simulink model "KUKA_coupled"  (R2021b)
settings: Solver=ode4  StartTime=0.0  StopTime=0.01  FixedStep=0.01  RelTol=1e-3  EnableMultiTasking=on
InitFcn:
  | % ************** Initiate forces
  | % f0=[0;0;0;0;0;0];
  | % f0=[0;0;0;0;0;0;0];
  | %f_0=[0;0;0];
  | %f_m=[0;0];
  | %f_e=[0;0;0;0;0;0];
  | %iota0=eye(6);
  | % ************** Initiate states
  | %q_m=[2;1];
  | %q_dot_m=[0;1];
  | %P=[0;0;0];
  | %V_I0=[0;0;0];
  | % ************** Load main
  | %run(Main.m)
StopFcn:
  | %format long
  | %table(out.qddot.data(:,1)',out.qddot_ref.data(1,:))
values from neighbouring files (symbols this model uses):
  diag_M = diagonalize(M_frak0, M_frak)    [Create_Robot.m]    (also in Main.m; Main__iiwa7.m; diagonalize.m = zeros(6*(n+1),6*(n+1)); test_C_Main.m)
  f_0 = [0;0;0]    [Create_Robot.m]    (also in Main.m; Main__iiwa7.m = [0;0;0;0;0;0]; test_C_Main.m)
  f_e = [0;0;0;0;0;0]    [Create_Robot.m]    (also in Main.m = [0;0;0]; Main__iiwa7.m; test_C_Main.m)
  f_m = [0;0]    [Create_Robot.m]    (also in Main.m; Main__iiwa7.m; test_C_Main.m)
  I0 = eye(3)*416.667    [Create_Robot.m]    (also in Main.m; Main__iiwa7.m = eye(3)*1.66667; test_C_Main.m)
  iota0 = [1 0 0; 0 1 0;zeros(3,3);0 0 1]    [Create_Robot.m]    (also in Main.m = [1 0 0 0 0 0; 0 1 0 0 0 0; 0 0 0 0 0 1]'; Main__iiwa7.m = eye(6,6); test_C_Main.m)
  m0 = 100    [Create_Robot.m]    (also in Main.m; Main__iiwa7.m = 10; test_C_Main.m)
  P = [0;0;0]    [Create_Robot.m]    (also in Main.m = M0*V_I0+M0m*q_dot_m; Main__iiwa7.m = M0*V_I0+M0m*q_dot_m; test_C_Main.m)
  q_dot_m = [0;0]    [Create_Robot.m]    (also in Main.m; Main__iiwa7.m; test_C_Main.m)
  q_m = [0;0]    [Create_Robot.m]    (also in Main.m = [0.2;0.4]; Main__iiwa7.m = [0.2;0.4]; test_C_Main.m = [1;0])
  sc_size = 5    [Main.m]    (also in Main__iiwa7.m = 1)
  X = [0 -x(3) x(2) ; x(3) 0 -x(1) ; -x(2) x(1) 0 ]    [skewsym.m]
  Xi_m_matrix = zeros(6*n,n)    [Create_Robot.m]    (also in Main.m; Main__iiwa7.m; test_C_Main.m)
undefined symbols (not defined in the file or in its folder): rho_0t, V_0t, Xi_m, Y, Z
libraries: sm_lib x87, nesl_utility x51, robotcorelib x2
(part 2 of 3)

== system KUKA_coupled/Space Manipulator1/joint//link2 ==
  iiwa_joint_2 : sm_lib/Joints/Revolute Joint  JointMode=Normal  SenseConstraintForce=off  SenseConstraintForceX=off  SenseConstraintForceY=off  SenseConstraintForceZ=off  SenseConstraintTorque=off  SenseConstraintTorqueX=off  SenseConstraintTorqueY=off  SenseConstraintTorqueZ=off  SenseTotalForce=off  SenseTotalForceX=off  SenseTotalForceY=off  SenseTotalForceZ=off  SenseTotalTorque=off  SenseTotalTorqueX=off  SenseTotalTorqueY=off  SenseTotalTorqueZ=off  CompositeWrenchDir=FollowerOnBase  CompositeWrenchFrame=BaseFrame  EquilibriumPosition=0  EquilibriumPositionUnits=deg  SpringStiffness=0  SpringStiffnessUnits=N*m/deg  DampingCoefficient=0.5  DampingCoefficientUnits=kg*m^2/(rad*s)  TorqueActuationMode=InputTorque  MotionActuationMode=ComputedMotion  SensePosition=on  SenseVelocity=on  SenseAcceleration=on  SenseTorqueForce=off  SenseLowerLimitTorqueForce=off  SenseUpperLimitTorqueForce=off  LowerLimitSpecify=on  LowerLimitBound=-2.09439510239  LowerLimitBoundUnits=rad  LowerLimitStiffness=1e4  LowerLimitStiffnessUnits=N*m/deg  LowerLimitDamping=10  LowerLimitDampingUnits=N*m/(deg/s)  LowerLimitTransitionRegionWidth=0.1  LowerLimitTransitionRegionWidthUnits=deg  UpperLimitSpecify=on  UpperLimitBound=2.09439510239  UpperLimitBoundUnits=rad  UpperLimitStiffness=1e4  UpperLimitStiffnessUnits=N*m/deg  UpperLimitDamping=10  UpperLimitDampingUnits=N*m/(deg/s)  UpperLimitTransitionRegionWidth=0.1  UpperLimitTransitionRegionWidthUnits=deg  PositionTargetSpecify=on  PositionTargetPriority=High  PositionTargetValue=1  PositionTargetValueUnits=rad  VelocityTargetSpecify=off  VelocityTargetPriority=High  VelocityTargetValue=0  VelocityTargetValueUnits=deg/s
  iiwa_link_2 : Subsystem
  b : PMIOPort  Side=Left
  F1 : PMIOPort  Port=2  Side=Right
  f2 : PMIOPort  Port=3  Side=Left
  q2 : PMIOPort  Port=4  Side=Right
  qd2 : PMIOPort  Port=5  Side=Right
  qdd2 : PMIOPort  Port=6  Side=Right
  connections:
  iiwa_joint_2/RConn3 -- qd2/RConn1
  iiwa_joint_2/RConn1 -- iiwa_link_2/LConn1
  F1/RConn1 -- iiwa_link_2/RConn1
  iiwa_joint_2/RConn4 -- qdd2/RConn1
  iiwa_joint_2/LConn1 -- b/RConn1
  f2/RConn1 -- iiwa_joint_2/LConn2
  iiwa_joint_2/RConn2 -- q2/RConn1

== system KUKA_coupled/Space Manipulator1/joint//link3 ==
  iiwa_joint_3 : sm_lib/Joints/Revolute Joint  JointMode=Normal  SenseConstraintForce=off  SenseConstraintForceX=off  SenseConstraintForceY=off  SenseConstraintForceZ=off  SenseConstraintTorque=off  SenseConstraintTorqueX=off  SenseConstraintTorqueY=off  SenseConstraintTorqueZ=off  SenseTotalForce=off  SenseTotalForceX=off  SenseTotalForceY=off  SenseTotalForceZ=off  SenseTotalTorque=off  SenseTotalTorqueX=off  SenseTotalTorqueY=off  SenseTotalTorqueZ=off  CompositeWrenchDir=FollowerOnBase  CompositeWrenchFrame=BaseFrame  EquilibriumPosition=0  EquilibriumPositionUnits=deg  SpringStiffness=0  SpringStiffnessUnits=N*m/deg  DampingCoefficient=0.5  DampingCoefficientUnits=kg*m^2/(rad*s)  TorqueActuationMode=InputTorque  MotionActuationMode=ComputedMotion  SensePosition=on  SenseVelocity=on  SenseAcceleration=on  SenseTorqueForce=off  SenseLowerLimitTorqueForce=off  SenseUpperLimitTorqueForce=off  LowerLimitSpecify=on  LowerLimitBound=-2.96705972839  LowerLimitBoundUnits=rad  LowerLimitStiffness=1e4  LowerLimitStiffnessUnits=N*m/deg  LowerLimitDamping=10  LowerLimitDampingUnits=N*m/(deg/s)  LowerLimitTransitionRegionWidth=0.1  LowerLimitTransitionRegionWidthUnits=deg  UpperLimitSpecify=on  UpperLimitBound=2.96705972839  UpperLimitBoundUnits=rad  UpperLimitStiffness=1e4  UpperLimitStiffnessUnits=N*m/deg  UpperLimitDamping=10  UpperLimitDampingUnits=N*m/(deg/s)  UpperLimitTransitionRegionWidth=0.1  UpperLimitTransitionRegionWidthUnits=deg  PositionTargetSpecify=off  PositionTargetPriority=High  PositionTargetValue=0  PositionTargetValueUnits=deg  VelocityTargetSpecify=off  VelocityTargetPriority=High  VelocityTargetValue=0  VelocityTargetValueUnits=deg/s
  iiwa_link_3 : Subsystem
  b : PMIOPort  Side=Left
  F1 : PMIOPort  Port=2  Side=Right
  f3 : PMIOPort  Port=3  Side=Left
  q3 : PMIOPort  Port=4  Side=Right
  qd3 : PMIOPort  Port=5  Side=Right
  qdd3 : PMIOPort  Port=6  Side=Right
  connections:
  iiwa_joint_3/RConn1 -- iiwa_link_3/LConn1
  iiwa_joint_3/RConn4 -- qdd3/RConn1
  iiwa_joint_3/RConn3 -- qd3/RConn1
  iiwa_joint_3/RConn2 -- q3/RConn1
  F1/RConn1 -- iiwa_link_3/RConn1
  f3/RConn1 -- iiwa_joint_3/LConn2
  iiwa_joint_3/LConn1 -- b/RConn1

== system KUKA_coupled/Space Manipulator1/joint//link4 ==
  iiwa_joint_4 : sm_lib/Joints/Revolute Joint  JointMode=Normal  SenseConstraintForce=off  SenseConstraintForceX=off  SenseConstraintForceY=off  SenseConstraintForceZ=off  SenseConstraintTorque=off  SenseConstraintTorqueX=off  SenseConstraintTorqueY=off  SenseConstraintTorqueZ=off  SenseTotalForce=off  SenseTotalForceX=off  SenseTotalForceY=off  SenseTotalForceZ=off  SenseTotalTorque=off  SenseTotalTorqueX=off  SenseTotalTorqueY=off  SenseTotalTorqueZ=off  CompositeWrenchDir=FollowerOnBase  CompositeWrenchFrame=BaseFrame  EquilibriumPosition=0  EquilibriumPositionUnits=deg  SpringStiffness=0  SpringStiffnessUnits=N*m/deg  DampingCoefficient=0.5  DampingCoefficientUnits=kg*m^2/(rad*s)  TorqueActuationMode=InputTorque  MotionActuationMode=ComputedMotion  SensePosition=on  SenseVelocity=on  SenseAcceleration=on  SenseTorqueForce=off  SenseLowerLimitTorqueForce=off  SenseUpperLimitTorqueForce=off  LowerLimitSpecify=on  LowerLimitBound=-2.09439510239  LowerLimitBoundUnits=rad  LowerLimitStiffness=1e4  LowerLimitStiffnessUnits=N*m/deg  LowerLimitDamping=10  LowerLimitDampingUnits=N*m/(deg/s)  LowerLimitTransitionRegionWidth=0.1  LowerLimitTransitionRegionWidthUnits=deg  UpperLimitSpecify=on  UpperLimitBound=2.09439510239  UpperLimitBoundUnits=rad  UpperLimitStiffness=1e4  UpperLimitStiffnessUnits=N*m/deg  UpperLimitDamping=10  UpperLimitDampingUnits=N*m/(deg/s)  UpperLimitTransitionRegionWidth=0.1  UpperLimitTransitionRegionWidthUnits=deg  PositionTargetSpecify=on  PositionTargetPriority=High  PositionTargetValue=1  PositionTargetValueUnits=rad  VelocityTargetSpecify=off  VelocityTargetPriority=High  VelocityTargetValue=0  VelocityTargetValueUnits=deg/s
  iiwa_link_4 : Subsystem
  b : PMIOPort  Side=Left
  F1 : PMIOPort  Port=2  Side=Right
  f4 : PMIOPort  Port=3  Side=Left
  q4 : PMIOPort  Port=4  Side=Right
  qd4 : PMIOPort  Port=5  Side=Right
  qd5 : PMIOPort  Port=6  Side=Right
  connections:
  iiwa_joint_4/RConn1 -- iiwa_link_4/LConn1
  iiwa_joint_4/RConn3 -- qd4/RConn1
  f4/RConn1 -- iiwa_joint_4/LConn2
  F1/RConn1 -- iiwa_link_4/RConn1
  iiwa_joint_4/RConn2 -- q4/RConn1
  iiwa_joint_4/LConn1 -- b/RConn1
  iiwa_joint_4/RConn4 -- qd5/RConn1

== system KUKA_coupled/Space Manipulator1/joint//link5 ==
  iiwa_joint_5 : sm_lib/Joints/Revolute Joint  JointMode=Normal  SenseConstraintForce=off  SenseConstraintForceX=off  SenseConstraintForceY=off  SenseConstraintForceZ=off  SenseConstraintTorque=off  SenseConstraintTorqueX=off  SenseConstraintTorqueY=off  SenseConstraintTorqueZ=off  SenseTotalForce=off  SenseTotalForceX=off  SenseTotalForceY=off  SenseTotalForceZ=off  SenseTotalTorque=off  SenseTotalTorqueX=off  SenseTotalTorqueY=off  SenseTotalTorqueZ=off  CompositeWrenchDir=FollowerOnBase  CompositeWrenchFrame=BaseFrame  EquilibriumPosition=0  EquilibriumPositionUnits=deg  SpringStiffness=0  SpringStiffnessUnits=N*m/deg  DampingCoefficient=0.5  DampingCoefficientUnits=kg*m^2/(rad*s)  TorqueActuationMode=InputTorque  MotionActuationMode=ComputedMotion  SensePosition=on  SenseVelocity=on  SenseAcceleration=on  SenseTorqueForce=off  SenseLowerLimitTorqueForce=off  SenseUpperLimitTorqueForce=off  LowerLimitSpecify=on  LowerLimitBound=-2.96705972839  LowerLimitBoundUnits=rad  LowerLimitStiffness=1e4  LowerLimitStiffnessUnits=N*m/deg  LowerLimitDamping=10  LowerLimitDampingUnits=N*m/(deg/s)  LowerLimitTransitionRegionWidth=0.1  LowerLimitTransitionRegionWidthUnits=deg  UpperLimitSpecify=on  UpperLimitBound=2.96705972839  UpperLimitBoundUnits=rad  UpperLimitStiffness=1e4  UpperLimitStiffnessUnits=N*m/deg  UpperLimitDamping=10  UpperLimitDampingUnits=N*m/(deg/s)  UpperLimitTransitionRegionWidth=0.1  UpperLimitTransitionRegionWidthUnits=deg  PositionTargetSpecify=off  PositionTargetPriority=High  PositionTargetValue=0  PositionTargetValueUnits=deg  VelocityTargetSpecify=off  VelocityTargetPriority=High  VelocityTargetValue=0  VelocityTargetValueUnits=deg/s
  iiwa_link_5 : Subsystem
  b : PMIOPort  Side=Left
  F1 : PMIOPort  Port=2  Side=Right
  f5 : PMIOPort  Port=3  Side=Left
  q5 : PMIOPort  Port=4  Side=Right
  qd5 : PMIOPort  Port=5  Side=Right
  qdd5 : PMIOPort  Port=6  Side=Right
  connections:
  iiwa_joint_5/LConn1 -- b/RConn1
  iiwa_joint_5/RConn2 -- q5/RConn1
  iiwa_joint_5/RConn4 -- qdd5/RConn1
  iiwa_joint_5/RConn1 -- iiwa_link_5/LConn1
  iiwa_joint_5/RConn3 -- qd5/RConn1
  f5/RConn1 -- iiwa_joint_5/LConn2
  F1/RConn1 -- iiwa_link_5/RConn1

== system KUKA_coupled/Space Manipulator1/joint//link6 ==
  iiwa_joint_6 : sm_lib/Joints/Revolute Joint  JointMode=Normal  SenseConstraintForce=off  SenseConstraintForceX=off  SenseConstraintForceY=off  SenseConstraintForceZ=off  SenseConstraintTorque=off  SenseConstraintTorqueX=off  SenseConstraintTorqueY=off  SenseConstraintTorqueZ=off  SenseTotalForce=off  SenseTotalForceX=off  SenseTotalForceY=off  SenseTotalForceZ=off  SenseTotalTorque=off  SenseTotalTorqueX=off  SenseTotalTorqueY=off  SenseTotalTorqueZ=off  CompositeWrenchDir=FollowerOnBase  CompositeWrenchFrame=BaseFrame  EquilibriumPosition=0  EquilibriumPositionUnits=deg  SpringStiffness=0  SpringStiffnessUnits=N*m/deg  DampingCoefficient=0.5  DampingCoefficientUnits=kg*m^2/(rad*s)  TorqueActuationMode=InputTorque  MotionActuationMode=ComputedMotion  SensePosition=on  SenseVelocity=on  SenseAcceleration=on  SenseTorqueForce=off  SenseLowerLimitTorqueForce=off  SenseUpperLimitTorqueForce=off  LowerLimitSpecify=on  LowerLimitBound=-2.09439510239  LowerLimitBoundUnits=rad  LowerLimitStiffness=1e4  LowerLimitStiffnessUnits=N*m/deg  LowerLimitDamping=10  LowerLimitDampingUnits=N*m/(deg/s)  LowerLimitTransitionRegionWidth=0.1  LowerLimitTransitionRegionWidthUnits=deg  UpperLimitSpecify=on  UpperLimitBound=2.09439510239  UpperLimitBoundUnits=rad  UpperLimitStiffness=1e4  UpperLimitStiffnessUnits=N*m/deg  UpperLimitDamping=10  UpperLimitDampingUnits=N*m/(deg/s)  UpperLimitTransitionRegionWidth=0.1  UpperLimitTransitionRegionWidthUnits=deg  PositionTargetSpecify=off  PositionTargetPriority=High  PositionTargetValue=0  PositionTargetValueUnits=deg  VelocityTargetSpecify=off  VelocityTargetPriority=High  VelocityTargetValue=0  VelocityTargetValueUnits=deg/s
  iiwa_link_6 : Subsystem
  b : PMIOPort  Side=Left
  F1 : PMIOPort  Port=2  Side=Right
  q6 : PMIOPort  Port=3  Side=Right
  f6 : PMIOPort  Port=4  Side=Left
  qd6 : PMIOPort  Port=5  Side=Right
  qdd6 : PMIOPort  Port=6  Side=Right
  connections:
  iiwa_joint_6/RConn1 -- iiwa_link_6/LConn1
  iiwa_joint_6/LConn1 -- b/RConn1
  F1/RConn1 -- iiwa_link_6/RConn1
  f6/RConn1 -- iiwa_joint_6/LConn2
  iiwa_joint_6/RConn4 -- qdd6/RConn1
  iiwa_joint_6/RConn3 -- qd6/RConn1
  iiwa_joint_6/RConn2 -- q6/RConn1

== system KUKA_coupled/Space Manipulator1/joint//link7 ==
  iiwa_joint_7 : sm_lib/Joints/Revolute Joint  JointMode=Normal  SenseConstraintForce=off  SenseConstraintForceX=off  SenseConstraintForceY=off  SenseConstraintForceZ=off  SenseConstraintTorque=off  SenseConstraintTorqueX=off  SenseConstraintTorqueY=off  SenseConstraintTorqueZ=off  SenseTotalForce=off  SenseTotalForceX=off  SenseTotalForceY=off  SenseTotalForceZ=off  SenseTotalTorque=off  SenseTotalTorqueX=off  SenseTotalTorqueY=off  SenseTotalTorqueZ=off  CompositeWrenchDir=FollowerOnBase  CompositeWrenchFrame=BaseFrame  EquilibriumPosition=0  EquilibriumPositionUnits=deg  SpringStiffness=0  SpringStiffnessUnits=N*m/deg  DampingCoefficient=0.5  DampingCoefficientUnits=kg*m^2/(rad*s)  TorqueActuationMode=InputTorque  MotionActuationMode=ComputedMotion  SensePosition=on  SenseVelocity=on  SenseAcceleration=on  SenseTorqueForce=off  SenseLowerLimitTorqueForce=off  SenseUpperLimitTorqueForce=off  LowerLimitSpecify=on  LowerLimitBound=-3.05432619099  LowerLimitBoundUnits=rad  LowerLimitStiffness=1e4  LowerLimitStiffnessUnits=N*m/deg  LowerLimitDamping=10  LowerLimitDampingUnits=N*m/(deg/s)  LowerLimitTransitionRegionWidth=0.1  LowerLimitTransitionRegionWidthUnits=deg  UpperLimitSpecify=on  UpperLimitBound=3.05432619099  UpperLimitBoundUnits=rad  UpperLimitStiffness=1e4  UpperLimitStiffnessUnits=N*m/deg  UpperLimitDamping=10  UpperLimitDampingUnits=N*m/(deg/s)  UpperLimitTransitionRegionWidth=0.1  UpperLimitTransitionRegionWidthUnits=deg  PositionTargetSpecify=off  PositionTargetPriority=High  PositionTargetValue=0  PositionTargetValueUnits=deg  VelocityTargetSpecify=off  VelocityTargetPriority=High  VelocityTargetValue=0  VelocityTargetValueUnits=deg/s
  iiwa_link_7 : Subsystem
  F2 : PMIOPort  Side=Right
  b : PMIOPort  Port=2  Side=Left
  F1 : PMIOPort  Port=3  Side=Right
  q7 : PMIOPort  Port=4  Side=Right
  f7 : PMIOPort  Port=5  Side=Left
  qd7 : PMIOPort  Port=6  Side=Right
  qdd7 : PMIOPort  Port=7  Side=Right
  connections:
  iiwa_joint_7/RConn1 -- iiwa_link_7/LConn1
  iiwa_joint_7/RConn4 -- qdd7/RConn1
  iiwa_joint_7/RConn2 -- q7/RConn1
  iiwa_joint_7/RConn3 -- qd7/RConn1
  f7/RConn1 -- iiwa_joint_7/LConn2
  F1/RConn1 -- iiwa_link_7/RConn2
  F2/RConn1 -- iiwa_link_7/RConn1
  iiwa_joint_7/LConn1 -- b/RConn1

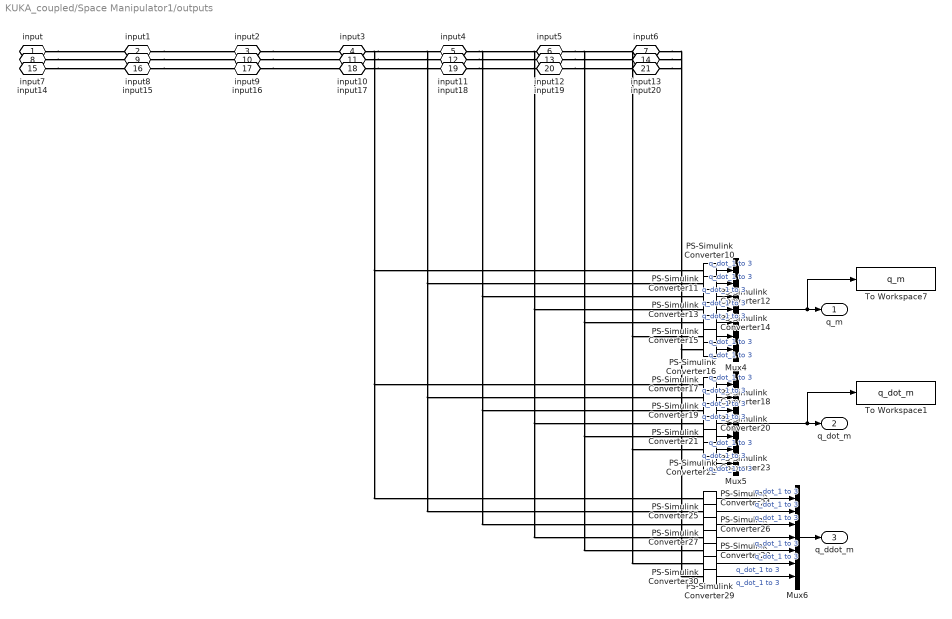
== system KUKA_coupled/Space Manipulator1/outputs ==
  Mux4 : Mux  Inputs=7
  Mux5 : Mux  Inputs=7
  Mux6 : Mux  Inputs=7
  PS-Simulink Converter{10..30} (21 alike) : nesl_utility/PS-Simulink Converter  PhysicalDomain=network_engine_domain  SubClassName=ps_output  LeftPortType=input  RightPortType=output  PseudoPeriodic=off  Frequencies=[]  Unit=inherit  AffineConversion=off
      settings: SourceProductBaseCode=PW,SS
  To Workspace1 : ToWorkspace  VariableName=q_dot_m  SampleTime=-1
  To Workspace7 : ToWorkspace  VariableName=q_m  SampleTime=-1
  input : PMIOPort  Side=Left
  input1 : PMIOPort  Port=2  Side=Left
  input2 : PMIOPort  Port=3  Side=Left
  input3 : PMIOPort  Port=4  Side=Left
  input4 : PMIOPort  Port=5  Side=Left
  input5 : PMIOPort  Port=6  Side=Left
  input6 : PMIOPort  Port=7  Side=Left
  input7 : PMIOPort  Port=8  Side=Left
  input8 : PMIOPort  Port=9  Side=Left
  input9 : PMIOPort  Port=10  Side=Left
  input10 : PMIOPort  Port=11  Side=Left
  input11 : PMIOPort  Port=12  Side=Left
  input12 : PMIOPort  Port=13  Side=Left
  input13 : PMIOPort  Port=14  Side=Left
  input14 : PMIOPort  Port=15  Side=Left
  input15 : PMIOPort  Port=16  Side=Left
  input16 : PMIOPort  Port=17  Side=Left
  input17 : PMIOPort  Port=18  Side=Left
  input18 : PMIOPort  Port=19  Side=Left
  input19 : PMIOPort  Port=20  Side=Left
  input20 : PMIOPort  Port=21  Side=Left
  q_m : Outport
  q_dot_m : Outport  Port=2
  q_ddot_m : Outport  Port=3
  wires:
  PS-Simulink Converter21/1 -> Mux5/5  "q_dot_1 to 3"
  PS-Simulink Converter12/1 -> Mux4/3  "q_dot_1 to 3"
  PS-Simulink Converter29/1 -> Mux6/6  "q_dot_1 to 3"
  PS-Simulink Converter14/1 -> Mux4/5  "q_dot_1 to 3"
  PS-Simulink Converter26/1 -> Mux6/3  "q_dot_1 to 3"
  PS-Simulink Converter17/1 -> Mux5/1  "q_dot_1 to 3"
  PS-Simulink Converter11/1 -> Mux4/2  "q_dot_1 to 3"
  PS-Simulink Converter25/1 -> Mux6/2  "q_dot_1 to 3"
  PS-Simulink Converter24/1 -> Mux6/1  "q_dot_1 to 3"
  PS-Simulink Converter10/1 -> Mux4/1  "q_dot_1 to 3"
  PS-Simulink Converter27/1 -> Mux6/4  "q_dot_1 to 3"
  PS-Simulink Converter28/1 -> Mux6/5  "q_dot_1 to 3"
  PS-Simulink Converter15/1 -> Mux4/6  "q_dot_1 to 3"
  PS-Simulink Converter16/1 -> Mux4/7  "q_dot_1 to 3"
  PS-Simulink Converter18/1 -> Mux5/2  "q_dot_1 to 3"
  PS-Simulink Converter30/1 -> Mux6/7  "q_dot_1 to 3"
  PS-Simulink Converter13/1 -> Mux4/4  "q_dot_1 to 3"
  PS-Simulink Converter22/1 -> Mux5/6  "q_dot_1 to 3"
  PS-Simulink Converter23/1 -> Mux5/7  "q_dot_1 to 3"
  PS-Simulink Converter20/1 -> Mux5/4  "q_dot_1 to 3"
  PS-Simulink Converter19/1 -> Mux5/3  "q_dot_1 to 3"
  Mux5/1 -> To Workspace1/1, q_dot_m/1
  Mux6/1 -> q_ddot_m/1
  Mux4/1 -> To Workspace7/1, q_m/1
  connections:
  input7/RConn1 -- PS-Simulink Converter17/LConn1
  input11/RConn1 -- PS-Simulink Converter21/LConn1
  input20/RConn1 -- PS-Simulink Converter30/LConn1
  input16/RConn1 -- PS-Simulink Converter26/LConn1
  input2/RConn1 -- PS-Simulink Converter12/LConn1
  input10/RConn1 -- PS-Simulink Converter20/LConn1
  input17/RConn1 -- PS-Simulink Converter27/LConn1
  input18/RConn1 -- PS-Simulink Converter28/LConn1
  input/RConn1 -- PS-Simulink Converter10/LConn1
  input19/RConn1 -- PS-Simulink Converter29/LConn1
  input5/RConn1 -- PS-Simulink Converter15/LConn1
  input14/RConn1 -- PS-Simulink Converter24/LConn1
  input6/RConn1 -- PS-Simulink Converter16/LConn1
  input9/RConn1 -- PS-Simulink Converter19/LConn1
  input8/RConn1 -- PS-Simulink Converter18/LConn1
  input15/RConn1 -- PS-Simulink Converter25/LConn1
  input12/RConn1 -- PS-Simulink Converter22/LConn1
  input13/RConn1 -- PS-Simulink Converter23/LConn1
  input1/RConn1 -- PS-Simulink Converter11/LConn1
  input4/RConn1 -- PS-Simulink Converter14/LConn1
  input3/RConn1 -- PS-Simulink Converter13/LConn1

== system KUKA_coupled/old model1/Inverse Dynamics ==
  f_m : Inport
  q_m q_dot_m : Inport  Port=2
  P : Inport  Port=3
  V : Inport  Port=4
  f_0 : Inport  Port=5
  Euler Poincare : Subsystem
  Internal Dynamics : Subsystem
  q_ddot : Outport
  P_dot : Outport  Port=2
  wires:
  f_m/1 -> Internal Dynamics/1(f_m)
  Internal Dynamics/1(q_ddot) -> q_ddot/1  "q_ddot"
  q_m q_dot_m/1 -> Internal Dynamics/2(q_m q_dot_m)
  f_0/1 -> Euler Poincare/3(f_0)
  Euler Poincare/1(P_dot) -> P_dot/1  "P_dot"
  V/1 -> Euler Poincare/2(V)
  P/1 -> Euler Poincare/1(P)

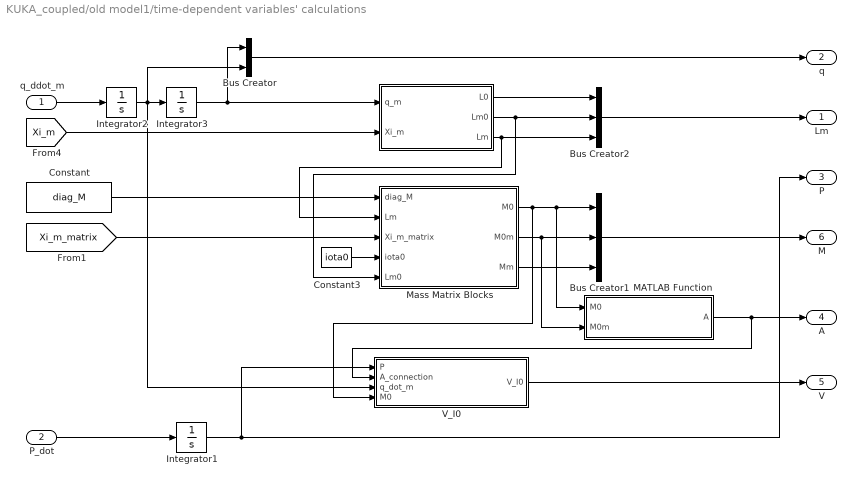
== system KUKA_coupled/old model1/time-dependent variables' calculations ==
  q_ddot_m : Inport
  P_dot : Inport  Port=2
  " " : MATLAB Function  TreatAsAtomicUnit=on
  Bus Creator : BusCreator  Inputs=2
  Bus Creator1 : BusCreator  Inputs=3
  Bus Creator2 : BusCreator  Inputs=3
  Constant : Constant  Value=diag_M  VectorParams1D=off
  Constant3 : Constant  Value=iota0  VectorParams1D=off
  Integrator1 : Integrator
  Integrator2 : Integrator
  Integrator3 : Integrator
  MATLAB Function : MATLAB Function  TreatAsAtomicUnit=on
  Mass Matrix Blocks : Subsystem
  V_I0 : MATLAB Function  TreatAsAtomicUnit=on
  Lm : Outport
  q : Outport  Port=2
  P : Outport  Port=3
  A : Outport  Port=4
  V : Outport  Port=5
  M : Outport  Port=6
  wires:
  Integrator2/1 -> V_I0/3(q_dot_m), Bus Creator/2, Integrator3/1
  q_ddot_m/1 -> Integrator2/1
  " "/1(L0) -> Bus Creator2/1
  " "/3(Lm) -> Mass Matrix Blocks/2(Lm), Bus Creator2/3
  " "/2(Lm0) -> Mass Matrix Blocks/5(Lm0), Bus Creator2/2
  Constant/1 -> Mass Matrix Blocks/1(diag_M)
  [Xi_m_matrix] -> Mass Matrix Blocks/3(Xi_m_matrix)
  [Xi_m] -> " "/2(Xi_m)
  Integrator3/1 -> Bus Creator/1, " "/1(q_m)
  Bus Creator/1 -> q/1
  Mass Matrix Blocks/1(M0) -> V_I0/4(M0), MATLAB Function/1(M0), Bus Creator1/1
  Mass Matrix Blocks/3(Mm) -> Bus Creator1/3
  Bus Creator1/1 -> M/1
  Mass Matrix Blocks/2(M0m) -> MATLAB Function/2(M0m), Bus Creator1/2
  MATLAB Function/1(A) -> V_I0/2(A_connection), A/1
  Constant3/1 -> Mass Matrix Blocks/4(iota0)
  Bus Creator2/1 -> Lm/1
  Integrator1/1 -> V_I0/1(P), P/1
  P_dot/1 -> Integrator1/1
  V_I0/1(V_I0) -> V/1

== system KUKA_coupled/time-dependent variables' calculations2/A_connection ==
  M0 : Inport
  M0m : Inport  Port=2
  Divide : Product  Inputs=/*  Multiplication=Matrix(*)
  Out1 : Outport
  wires:
  M0/1 -> Divide/1
  Divide/1 -> Out1/1
  M0m/1 -> Divide/2

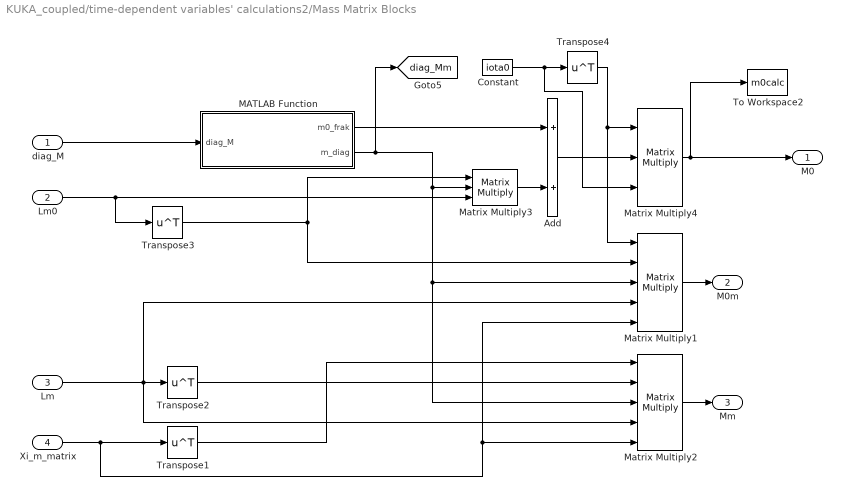
== system KUKA_coupled/time-dependent variables' calculations2/Mass Matrix Blocks ==
  diag_M : Inport
  Lm0 : Inport  Port=2
  Lm : Inport  Port=3
  Xi_m_matrix : Inport  Port=4
  Add : Sum
  Constant : Constant  Value=iota0
  MATLAB Function : MATLAB Function  TreatAsAtomicUnit=on
  Matrix Multiply1 : Product  Inputs=5  Multiplication=Matrix(*)
  Matrix Multiply2 : Product  Inputs=5  Multiplication=Matrix(*)
  Matrix Multiply3 : Product  Inputs=3  Multiplication=Matrix(*)
  Matrix Multiply4 : Product  Inputs=3  Multiplication=Matrix(*)
  To Workspace2 : ToWorkspace  VariableName=m0calc  SaveFormat=Timeseries  SampleTime=-1
  Transpose{1..4} (4 alike) : Math  Operator=transpose  SaturateOnIntegerOverflow=on
  M0 : Outport
  M0m : Outport  Port=2
  Mm : Outport  Port=3
  tag scope: diag_Mm=global
  wires:
  Matrix Multiply2/1 -> Mm/1
  Xi_m_matrix/1 -> Matrix Multiply1/5, Matrix Multiply2/5, Transpose1/1
  diag_M/1 -> MATLAB Function/1(diag_M)
  Lm/1 -> Matrix Multiply1/4, Matrix Multiply2/4, Transpose2/1
  Transpose1/1 -> Matrix Multiply2/1
  Transpose2/1 -> Matrix Multiply2/2
  MATLAB Function/1(m0_frak) -> Add/1
  MATLAB Function/2(m_diag) -> Matrix Multiply3/2, Matrix Multiply1/3, Matrix Multiply2/3, [diag_Mm]
  Matrix Multiply1/1 -> M0m/1
  Add/1 -> Matrix Multiply4/2
  Matrix Multiply3/1 -> Add/2
  Lm0/1 -> Transpose3/1, Matrix Multiply3/3
  Transpose3/1 -> Matrix Multiply3/1, Matrix Multiply1/2
  Constant/1 -> Matrix Multiply4/3, Transpose4/1
  Transpose4/1 -> Matrix Multiply1/1, Matrix Multiply4/1
  Matrix Multiply4/1 -> To Workspace2/1, M0/1

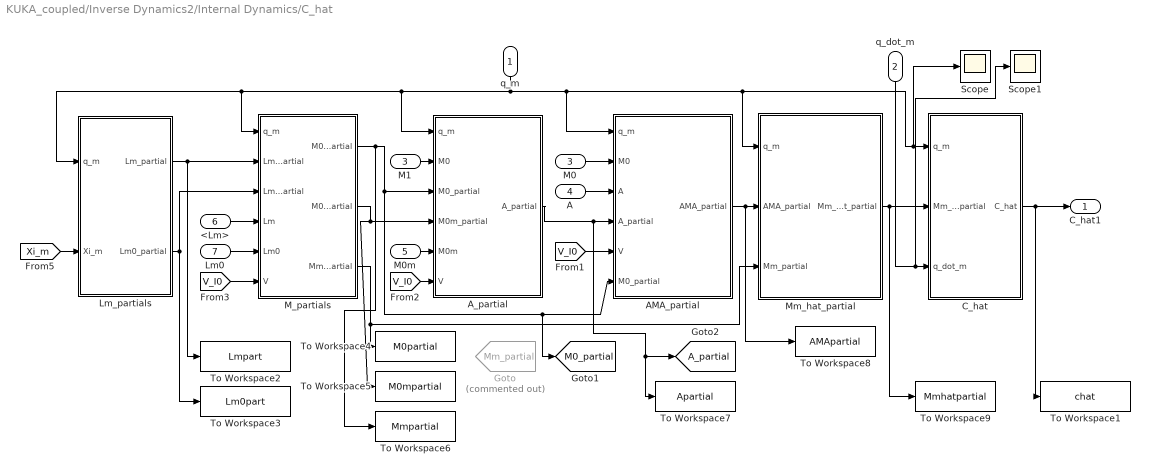
== system KUKA_coupled/Inverse Dynamics2/Internal Dynamics/C_hat ==
  q_m : Inport
  q_dot_m : Inport  Port=2
  M0 : Inport  Port=3
  A : Inport  Port=4
  M0m : Inport  Port=5
  <Lm> : Inport  Port=6
  Lm0 : Inport  Port=7
  AMA_partial : MATLAB Function  TreatAsAtomicUnit=on
  A_partial : MATLAB Function  TreatAsAtomicUnit=on
  C_hat : MATLAB Function  TreatAsAtomicUnit=on
  Goto : Goto  Commented=on  GotoTag=Mm_partial  TagVisibility=global
  Lm_partials : Subsystem
  M1 : InportShadow  Port=3
  M_partials : Subsystem
  Mm_hat_partial : MATLAB Function  TreatAsAtomicUnit=on
  Scope : Scope
  Scope1 : Scope
  To Workspace1 : ToWorkspace  VariableName=chat  SaveFormat=Timeseries  SampleTime=-1
  To Workspace2 : ToWorkspace  VariableName=Lmpart  SaveFormat=Timeseries  SampleTime=-1
  To Workspace3 : ToWorkspace  VariableName=Lm0part  SaveFormat=Timeseries  SampleTime=-1
  To Workspace4 : ToWorkspace  VariableName=M0partial  SaveFormat=Timeseries  SampleTime=-1
  To Workspace5 : ToWorkspace  VariableName=M0mpartial  SaveFormat=Timeseries  SampleTime=-1
  To Workspace6 : ToWorkspace  VariableName=Mmpartial  SaveFormat=Timeseries  SampleTime=-1
  To Workspace7 : ToWorkspace  VariableName=Apartial  SaveFormat=Timeseries  SampleTime=-1
  To Workspace8 : ToWorkspace  VariableName=AMApartial  SaveFormat=Timeseries  SampleTime=-1
  To Workspace9 : ToWorkspace  VariableName=Mmhatpartial  SaveFormat=Timeseries  SampleTime=-1
  C_hat1 : Outport
  tag scope: A_partial=global, M0_partial=global
  wires:
  C_hat/1(C_hat) -> To Workspace1/1, C_hat1/1
  q_m/1 -> AMA_partial/1(q_m), Mm_hat_partial/1(q_m), Scope/1, C_hat/1(q_m), A_partial/1(q_m), Lm_partials/1(q_m), M_partials/1(q_m)
  q_dot_m/1 -> Scope1/1, C_hat/3(q_dot_m)
  <Lm>/1 -> M_partials/4(Lm)
  [Xi_m] -> Lm_partials/2(Xi_m)
  Lm_partials/1(Lm_partial) -> To Workspace2/1, M_partials/2(Lm_partial)
  M_partials/3(Mm_partial) -> To Workspace4/1, Mm_hat_partial/3(Mm_partial)
  Mm_hat_partial/1(Mm_hat_partial) -> To Workspace9/1, C_hat/2(Mm_hat_partial)
  AMA_partial/1(AMA_partial) -> To Workspace8/1, Mm_hat_partial/2(AMA_partial)
  M0/1 -> AMA_partial/2(M0)
  M_partials/1(M0_partial) -> To Workspace6/1, [M0_partial], AMA_partial/6(M0_partial), A_partial/3(M0_partial)
  A/1 -> AMA_partial/3(A)
  A_partial/1(A_partial) -> To Workspace7/1, [A_partial], AMA_partial/4(A_partial)
  [V_I0] -> AMA_partial/5(V)
  M1/1 -> A_partial/2(M0)
  M0m/1 -> A_partial/5(M0m)
  [V_I0] -> A_partial/6(V)
  M_partials/2(M0m_partial) -> To Workspace5/1, A_partial/4(M0m_partial)
  Lm_partials/2(Lm0_partial) -> M_partials/3(Lm0_partial), To Workspace3/1
  Lm0/1 -> M_partials/5(Lm0)
  [V_I0] -> M_partials/6(V)

== system KUKA_coupled/Inverse Dynamics2/Internal Dynamics/N_hat ==
  q_m : Inport
  q_dot_m : Inport  Port=2
  A : Inport  Port=3
  P : Inport  Port=4
  M0 : Inport  Port=5
  Constant : Constant  Value=iota0
  Matrix Multiply : Product  Multiplication=Matrix(*)
  N_hat : MATLAB Function  TreatAsAtomicUnit=on
  To Workspace : ToWorkspace  VariableName=N_firstpart  SaveFormat=Timeseries  SampleTime=-1
  N_hat1 : Outport
  wires:
  P/1 -> Matrix Multiply/2, N_hat/5(P)
  [M0_partial] -> N_hat/6(M0_partial)
  N_hat/1(N_hat_temp) -> To Workspace/1, Matrix Multiply/1
  q_m/1 -> N_hat/1(q_m)
  q_dot_m/1 -> N_hat/2(q_dot_m)
  [V_I0] -> N_hat/4(V)
  A/1 -> N_hat/3(A)
  [A_partial] -> N_hat/7(A_partial)
  Constant/1 -> N_hat/8(iota0)
  Matrix Multiply/1 -> N_hat1/1
  M0/1 -> N_hat/9(M0)

== system KUKA_coupled/Space Manipulator1/fixed base/iiwa_link_0 ==
  Inertia : sm_lib/Body Elements/Inertia  InertiaType=Custom  Mass=5  MassUnits=kg  CenterOfMass=[0, 0, 0]  CenterOfMassUnits=m  MomentsOfInertia=[0.05, 0.06, 0.03]  MomentsOfInertiaUnits=kg*m^2  ProductsOfInertia=[0, 0, 0]  ProductsOfInertiaUnits=kg*m^2  GraphicType=None  MarkerShape=Inertia  MarkerSize=20  GraphicVisPropType=SimpleVisualProperties  GraphicDiffuseColor=[0.5 0.5 0.5]  GraphicSpecularColor=[0.5 0.5 0.5 1.0]  GraphicAmbientColor=[0.15 0.15 0.15 1.0]  GraphicEmissiveColor=[0.0 0.0 0.0 1.0]  GraphicShininess=75  GraphicOpacity=1.0
  InertiaOriginTransform : sm_lib/Frames and Transforms/Rigid Transform  TranslationMethod=Cartesian  TranslationStandardOffset=0  TranslationLengthUnit=m  TranslationStandardAxis=+Z  TranslationCartesianOffset=[-0.1, 0, 0.07000000000000001]  TranslationROffset=0  TranslationROffsetUnits=m  TranslationZOffset=0  TranslationZOffsetUnits=m  TranslationThetaOffset=0  TranslationThetaOffsetUnits=deg  RotationMethod=RotationSequence  RotationAngleUnits=deg  RotationStandardAxis=+Z  RotationAngle=0.0  RotationArbitraryAxis=[0 0 1]  FollAlignAxisA=+X  BaseAlignAxisA=+Y  FollAlignAxisB=+Y  BaseAlignAxisB=+Z  RotationSequenceAxes=BaseAxes  RotationSequence=XYZ  RotationSequenceAngles=[0, 0, 0]  RotationSequenceAnglesUnits=rad  RotationMatrix=[1 0 0; 0 1 0; 0 0 1]
  ReferenceFrame : sm_lib/Frames and Transforms/Reference Frame
  Visual : sm_lib/Body Elements/File Solid  ExtGeomFileName=iiwa_description/meshes/iiwa7/visual/link_0.stl  UnitType=Custom  ExtGeomFileUnits=m  StepReaderType=HEX  ExportConvexHullGeometry=off  InertiaType=Custom  Mass=0  MassUnits=kg  CenterOfMass=[0, 0, 0]  CenterOfMassUnits=m  MomentsOfInertia=[0, 0, 0]  MomentsOfInertiaUnits=kg*m^2  ProductsOfInertia=[0, 0, 0]  ProductsOfInertiaUnits=kg*m^2  BasedOnType=DensityFromFile  Density=1000  DensityUnits=kg/m^3  DoExposeReferenceFrame=on  SerializedFrames=<Frames/>  GraphicType=FromGeometry  MarkerShape=Sphere  MarkerSize=10  GraphicVisPropType=SimpleVisualProperties  GraphicDiffuseColor=[0.4, 0.4, 0.4]  GraphicSpecularColor=[0.5 0.5 0.5 1.0]  GraphicAmbientColor=[0.15 0.15 0.15 1.0]  GraphicEmissiveColor=[0.0 0.0 0.0 1.0]  GraphicShininess=75  GraphicOpacity=1
  VisualOriginTransform : sm_lib/Frames and Transforms/Rigid Transform  TranslationMethod=Cartesian  TranslationStandardOffset=0  TranslationLengthUnit=m  TranslationStandardAxis=+Z  TranslationCartesianOffset=[0, 0, 0]  TranslationROffset=0  TranslationROffsetUnits=m  TranslationZOffset=0  TranslationZOffsetUnits=m  TranslationThetaOffset=0  TranslationThetaOffsetUnits=deg  RotationMethod=RotationSequence  RotationAngleUnits=deg  RotationStandardAxis=+Z  RotationAngle=0.0  RotationArbitraryAxis=[0 0 1]  FollAlignAxisA=+X  BaseAlignAxisA=+Y  FollAlignAxisB=+Y  BaseAlignAxisB=+Z  RotationSequenceAxes=BaseAxes  RotationSequence=XYZ  RotationSequenceAngles=[0, 0, 0]  RotationSequenceAnglesUnits=rad  RotationMatrix=[1 0 0; 0 1 0; 0 0 1]
  iiwa_joint_1_AxisTransform : sm_lib/Frames and Transforms/Rigid Transform  TranslationMethod=Cartesian  TranslationStandardOffset=0  TranslationLengthUnit=m  TranslationStandardAxis=+Z  TranslationCartesianOffset=[0, 0, 0]  TranslationROffset=0  TranslationROffsetUnits=m  TranslationZOffset=0  TranslationZOffsetUnits=m  TranslationThetaOffset=0  TranslationThetaOffsetUnits=deg  RotationMethod=ArbitraryAxis  RotationAngleUnits=rad  RotationStandardAxis=+Z  RotationAngle=0  RotationArbitraryAxis=[1, 0, 0]  FollAlignAxisA=+X  BaseAlignAxisA=+Y  FollAlignAxisB=+Y  BaseAlignAxisB=+Z  RotationSequenceAxes=FollowerAxes  RotationSequence=XYX  RotationSequenceAngles=[0 0 0]  RotationSequenceAnglesUnits=deg  RotationMatrix=[1 0 0; 0 1 0; 0 0 1]
  iiwa_joint_1_OriginTransform : sm_lib/Frames and Transforms/Rigid Transform  TranslationMethod=Cartesian  TranslationStandardOffset=0  TranslationLengthUnit=m  TranslationStandardAxis=+Z  TranslationCartesianOffset=[0, 0, 0.02]  TranslationROffset=0  TranslationROffsetUnits=m  TranslationZOffset=0  TranslationZOffsetUnits=m  TranslationThetaOffset=0  TranslationThetaOffsetUnits=deg  RotationMethod=RotationSequence  RotationAngleUnits=deg  RotationStandardAxis=+Z  RotationAngle=0.0  RotationArbitraryAxis=[0 0 1]  FollAlignAxisA=+X  BaseAlignAxisA=+Y  FollAlignAxisB=+Y  BaseAlignAxisB=+Z  RotationSequenceAxes=BaseAxes  RotationSequence=XYZ  RotationSequenceAngles=[0, 0, 0]  RotationSequenceAnglesUnits=rad  RotationMatrix=[1 0 0; 0 1 0; 0 0 1]
  F : PMIOPort  Side=Left
  F1 : PMIOPort  Port=2  Side=Right
  connections:
  Inertia/RConn1 -- InertiaOriginTransform/RConn1
  InertiaOriginTransform/LConn1 -- ReferenceFrame/RConn1 -- F/RConn1 -- VisualOriginTransform/LConn1 -- iiwa_joint_1_OriginTransform/LConn1
  Visual/RConn1 -- VisualOriginTransform/RConn1
  iiwa_joint_1_AxisTransform/RConn1 -- F1/RConn1
  iiwa_joint_1_AxisTransform/LConn1 -- iiwa_joint_1_OriginTransform/RConn1

== system KUKA_coupled/Space Manipulator1/join//link 1/iiwa_link_1 ==
  Inertia : sm_lib/Body Elements/Inertia  InertiaType=Custom  Mass=3.4525  MassUnits=kg  CenterOfMass=[0, 0, 0]  CenterOfMassUnits=m  MomentsOfInertia=[0.02183, 0.007703, 0.02083]  MomentsOfInertiaUnits=kg*m^2  ProductsOfInertia=[-0.003887, 0, 0]  ProductsOfInertiaUnits=kg*m^2  GraphicType=None  MarkerShape=Inertia  MarkerSize=20  GraphicVisPropType=SimpleVisualProperties  GraphicDiffuseColor=[0.5 0.5 0.5]  GraphicSpecularColor=[0.5 0.5 0.5 1.0]  GraphicAmbientColor=[0.15 0.15 0.15 1.0]  GraphicEmissiveColor=[0.0 0.0 0.0 1.0]  GraphicShininess=75  GraphicOpacity=1.0
  InertiaOriginTransform : sm_lib/Frames and Transforms/Rigid Transform  TranslationMethod=Cartesian  TranslationStandardOffset=0  TranslationLengthUnit=m  TranslationStandardAxis=+Z  TranslationCartesianOffset=[0, -0.03, 0.12]  TranslationROffset=0  TranslationROffsetUnits=m  TranslationZOffset=0  TranslationZOffsetUnits=m  TranslationThetaOffset=0  TranslationThetaOffsetUnits=deg  RotationMethod=RotationSequence  RotationAngleUnits=deg  RotationStandardAxis=+Z  RotationAngle=0.0  RotationArbitraryAxis=[0 0 1]  FollAlignAxisA=+X  BaseAlignAxisA=+Y  FollAlignAxisB=+Y  BaseAlignAxisB=+Z  RotationSequenceAxes=BaseAxes  RotationSequence=XYZ  RotationSequenceAngles=[0, 0, 0]  RotationSequenceAnglesUnits=rad  RotationMatrix=[1 0 0; 0 1 0; 0 0 1]
  ReferenceFrame : sm_lib/Frames and Transforms/Reference Frame
  Visual : sm_lib/Body Elements/File Solid  ExtGeomFileName=iiwa_description/meshes/iiwa7/visual/link_1.stl  UnitType=Custom  ExtGeomFileUnits=m  StepReaderType=HEX  ExportConvexHullGeometry=off  InertiaType=Custom  Mass=0  MassUnits=kg  CenterOfMass=[0, 0, 0]  CenterOfMassUnits=m  MomentsOfInertia=[0, 0, 0]  MomentsOfInertiaUnits=kg*m^2  ProductsOfInertia=[0, 0, 0]  ProductsOfInertiaUnits=kg*m^2  BasedOnType=DensityFromFile  Density=1000  DensityUnits=kg/m^3  DoExposeReferenceFrame=on  SerializedFrames=<Frames/>  GraphicType=FromGeometry  MarkerShape=Sphere  MarkerSize=10  GraphicVisPropType=SimpleVisualProperties  GraphicDiffuseColor=[1, 0.423529411765, 0.0392156862745]  GraphicSpecularColor=[0.5 0.5 0.5 1.0]  GraphicAmbientColor=[0.15 0.15 0.15 1.0]  GraphicEmissiveColor=[0.0 0.0 0.0 1.0]  GraphicShininess=75  GraphicOpacity=1
  VisualOriginTransform : sm_lib/Frames and Transforms/Rigid Transform  TranslationMethod=Cartesian  TranslationStandardOffset=0  TranslationLengthUnit=m  TranslationStandardAxis=+Z  TranslationCartesianOffset=[0, 0, 0]  TranslationROffset=0  TranslationROffsetUnits=m  TranslationZOffset=0  TranslationZOffsetUnits=m  TranslationThetaOffset=0  TranslationThetaOffsetUnits=deg  RotationMethod=RotationSequence  RotationAngleUnits=deg  RotationStandardAxis=+Z  RotationAngle=0.0  RotationArbitraryAxis=[0 0 1]  FollAlignAxisA=+X  BaseAlignAxisA=+Y  FollAlignAxisB=+Y  BaseAlignAxisB=+Z  RotationSequenceAxes=BaseAxes  RotationSequence=XYZ  RotationSequenceAngles=[0, 0, 0]  RotationSequenceAnglesUnits=rad  RotationMatrix=[1 0 0; 0 1 0; 0 0 1]
  iiwa_joint_1_AxisInvTransform : sm_lib/Frames and Transforms/Rigid Transform  TranslationMethod=Cartesian  TranslationStandardOffset=0  TranslationLengthUnit=m  TranslationStandardAxis=+Z  TranslationCartesianOffset=[0, 0, 0]  TranslationROffset=0  TranslationROffsetUnits=m  TranslationZOffset=0  TranslationZOffsetUnits=m  TranslationThetaOffset=0  TranslationThetaOffsetUnits=deg  RotationMethod=ArbitraryAxis  RotationAngleUnits=rad  RotationStandardAxis=+Z  RotationAngle=0  RotationArbitraryAxis=[1, 0, 0]  FollAlignAxisA=+X  BaseAlignAxisA=+Y  FollAlignAxisB=+Y  BaseAlignAxisB=+Z  RotationSequenceAxes=FollowerAxes  RotationSequence=XYX  RotationSequenceAngles=[0 0 0]  RotationSequenceAnglesUnits=deg  RotationMatrix=[1 0 0; 0 1 0; 0 0 1]
  iiwa_joint_2_AxisTransform : sm_lib/Frames and Transforms/Rigid Transform  TranslationMethod=Cartesian  TranslationStandardOffset=0  TranslationLengthUnit=m  TranslationStandardAxis=+Z  TranslationCartesianOffset=[0, 0, 0]  TranslationROffset=0  TranslationROffsetUnits=m  TranslationZOffset=0  TranslationZOffsetUnits=m  TranslationThetaOffset=0  TranslationThetaOffsetUnits=deg  RotationMethod=ArbitraryAxis  RotationAngleUnits=rad  RotationStandardAxis=+Z  RotationAngle=0  RotationArbitraryAxis=[1, 0, 0]  FollAlignAxisA=+X  BaseAlignAxisA=+Y  FollAlignAxisB=+Y  BaseAlignAxisB=+Z  RotationSequenceAxes=FollowerAxes  RotationSequence=XYX  RotationSequenceAngles=[0 0 0]  RotationSequenceAnglesUnits=deg  RotationMatrix=[1 0 0; 0 1 0; 0 0 1]
  iiwa_joint_2_OriginTransform : sm_lib/Frames and Transforms/Rigid Transform  TranslationMethod=Cartesian  TranslationStandardOffset=0  TranslationLengthUnit=m  TranslationStandardAxis=+Z  TranslationCartesianOffset=[0, 0, 0.19]  TranslationROffset=0  TranslationROffsetUnits=m  TranslationZOffset=0  TranslationZOffsetUnits=m  TranslationThetaOffset=0  TranslationThetaOffsetUnits=deg  RotationMethod=RotationSequence  RotationAngleUnits=deg  RotationStandardAxis=+Z  RotationAngle=0.0  RotationArbitraryAxis=[0 0 1]  FollAlignAxisA=+X  BaseAlignAxisA=+Y  FollAlignAxisB=+Y  BaseAlignAxisB=+Z  RotationSequenceAxes=BaseAxes  RotationSequence=XYZ  RotationSequenceAngles=[1.57079632679, 0, 3.14159265359]  RotationSequenceAnglesUnits=rad  RotationMatrix=[1 0 0; 0 1 0; 0 0 1]
  F : PMIOPort  Side=Left
  F1 : PMIOPort  Port=2  Side=Right
  connections:
  Inertia/RConn1 -- InertiaOriginTransform/RConn1
  InertiaOriginTransform/LConn1 -- iiwa_joint_1_AxisInvTransform/LConn1 -- iiwa_joint_2_OriginTransform/LConn1 -- VisualOriginTransform/LConn1 -- ReferenceFrame/RConn1
  Visual/RConn1 -- VisualOriginTransform/RConn1
  iiwa_joint_1_AxisInvTransform/RConn1 -- F/RConn1
  iiwa_joint_2_AxisTransform/RConn1 -- F1/RConn1
  iiwa_joint_2_AxisTransform/LConn1 -- iiwa_joint_2_OriginTransform/RConn1

== system KUKA_coupled/Space Manipulator1/joint//link2/iiwa_link_2 ==
  Inertia : sm_lib/Body Elements/Inertia  InertiaType=Custom  Mass=3.4821  MassUnits=kg  CenterOfMass=[0, 0, 0]  CenterOfMassUnits=m  MomentsOfInertia=[0.02076, 0.02179, 0.00779]  MomentsOfInertiaUnits=kg*m^2  ProductsOfInertia=[0, -0.003626, 0]  ProductsOfInertiaUnits=kg*m^2  GraphicType=None  MarkerShape=Inertia  MarkerSize=20  GraphicVisPropType=SimpleVisualProperties  GraphicDiffuseColor=[0.5 0.5 0.5]  GraphicSpecularColor=[0.5 0.5 0.5 1.0]  GraphicAmbientColor=[0.15 0.15 0.15 1.0]  GraphicEmissiveColor=[0.0 0.0 0.0 1.0]  GraphicShininess=75  GraphicOpacity=1.0
  InertiaOriginTransform : sm_lib/Frames and Transforms/Rigid Transform  TranslationMethod=Cartesian  TranslationStandardOffset=0  TranslationLengthUnit=m  TranslationStandardAxis=+Z  TranslationCartesianOffset=[0.0003, 0.059, 0.042]  TranslationROffset=0  TranslationROffsetUnits=m  TranslationZOffset=0  TranslationZOffsetUnits=m  TranslationThetaOffset=0  TranslationThetaOffsetUnits=deg  RotationMethod=RotationSequence  RotationAngleUnits=deg  RotationStandardAxis=+Z  RotationAngle=0.0  RotationArbitraryAxis=[0 0 1]  FollAlignAxisA=+X  BaseAlignAxisA=+Y  FollAlignAxisB=+Y  BaseAlignAxisB=+Z  RotationSequenceAxes=BaseAxes  RotationSequence=XYZ  RotationSequenceAngles=[0, 0, 0]  RotationSequenceAnglesUnits=rad  RotationMatrix=[1 0 0; 0 1 0; 0 0 1]
  ReferenceFrame : sm_lib/Frames and Transforms/Reference Frame
  Visual : sm_lib/Body Elements/File Solid  ExtGeomFileName=iiwa_description/meshes/iiwa7/visual/link_2.stl  UnitType=Custom  ExtGeomFileUnits=m  StepReaderType=HEX  ExportConvexHullGeometry=off  InertiaType=Custom  Mass=0  MassUnits=kg  CenterOfMass=[0, 0, 0]  CenterOfMassUnits=m  MomentsOfInertia=[0, 0, 0]  MomentsOfInertiaUnits=kg*m^2  ProductsOfInertia=[0, 0, 0]  ProductsOfInertiaUnits=kg*m^2  BasedOnType=DensityFromFile  Density=1000  DensityUnits=kg/m^3  DoExposeReferenceFrame=on  SerializedFrames=<Frames/>  GraphicType=FromGeometry  MarkerShape=Sphere  MarkerSize=10  GraphicVisPropType=SimpleVisualProperties  GraphicDiffuseColor=[1, 0.423529411765, 0.0392156862745]  GraphicSpecularColor=[0.5 0.5 0.5 1.0]  GraphicAmbientColor=[0.15 0.15 0.15 1.0]  GraphicEmissiveColor=[0.0 0.0 0.0 1.0]  GraphicShininess=75  GraphicOpacity=1
  VisualOriginTransform : sm_lib/Frames and Transforms/Rigid Transform  TranslationMethod=Cartesian  TranslationStandardOffset=0  TranslationLengthUnit=m  TranslationStandardAxis=+Z  TranslationCartesianOffset=[0, 0, 0]  TranslationROffset=0  TranslationROffsetUnits=m  TranslationZOffset=0  TranslationZOffsetUnits=m  TranslationThetaOffset=0  TranslationThetaOffsetUnits=deg  RotationMethod=RotationSequence  RotationAngleUnits=deg  RotationStandardAxis=+Z  RotationAngle=0.0  RotationArbitraryAxis=[0 0 1]  FollAlignAxisA=+X  BaseAlignAxisA=+Y  FollAlignAxisB=+Y  BaseAlignAxisB=+Z  RotationSequenceAxes=BaseAxes  RotationSequence=XYZ  RotationSequenceAngles=[0, 0, 0]  RotationSequenceAnglesUnits=rad  RotationMatrix=[1 0 0; 0 1 0; 0 0 1]
  iiwa_joint_2_AxisInvTransform : sm_lib/Frames and Transforms/Rigid Transform  TranslationMethod=Cartesian  TranslationStandardOffset=0  TranslationLengthUnit=m  TranslationStandardAxis=+Z  TranslationCartesianOffset=[0, 0, 0]  TranslationROffset=0  TranslationROffsetUnits=m  TranslationZOffset=0  TranslationZOffsetUnits=m  TranslationThetaOffset=0  TranslationThetaOffsetUnits=deg  RotationMethod=ArbitraryAxis  RotationAngleUnits=rad  RotationStandardAxis=+Z  RotationAngle=0  RotationArbitraryAxis=[1, 0, 0]  FollAlignAxisA=+X  BaseAlignAxisA=+Y  FollAlignAxisB=+Y  BaseAlignAxisB=+Z  RotationSequenceAxes=FollowerAxes  RotationSequence=XYX  RotationSequenceAngles=[0 0 0]  RotationSequenceAnglesUnits=deg  RotationMatrix=[1 0 0; 0 1 0; 0 0 1]
  iiwa_joint_3_AxisTransform : sm_lib/Frames and Transforms/Rigid Transform  TranslationMethod=Cartesian  TranslationStandardOffset=0  TranslationLengthUnit=m  TranslationStandardAxis=+Z  TranslationCartesianOffset=[0, 0, 0]  TranslationROffset=0  TranslationROffsetUnits=m  TranslationZOffset=0  TranslationZOffsetUnits=m  TranslationThetaOffset=0  TranslationThetaOffsetUnits=deg  RotationMethod=ArbitraryAxis  RotationAngleUnits=rad  RotationStandardAxis=+Z  RotationAngle=0  RotationArbitraryAxis=[1, 0, 0]  FollAlignAxisA=+X  BaseAlignAxisA=+Y  FollAlignAxisB=+Y  BaseAlignAxisB=+Z  RotationSequenceAxes=FollowerAxes  RotationSequence=XYX  RotationSequenceAngles=[0 0 0]  RotationSequenceAnglesUnits=deg  RotationMatrix=[1 0 0; 0 1 0; 0 0 1]
  iiwa_joint_3_OriginTransform : sm_lib/Frames and Transforms/Rigid Transform  TranslationMethod=Cartesian  TranslationStandardOffset=0  TranslationLengthUnit=m  TranslationStandardAxis=+Z  TranslationCartesianOffset=[0, 0.21, 0]  TranslationROffset=0  TranslationROffsetUnits=m  TranslationZOffset=0  TranslationZOffsetUnits=m  TranslationThetaOffset=0  TranslationThetaOffsetUnits=deg  RotationMethod=RotationSequence  RotationAngleUnits=deg  RotationStandardAxis=+Z  RotationAngle=0.0  RotationArbitraryAxis=[0 0 1]  FollAlignAxisA=+X  BaseAlignAxisA=+Y  FollAlignAxisB=+Y  BaseAlignAxisB=+Z  RotationSequenceAxes=BaseAxes  RotationSequence=XYZ  RotationSequenceAngles=[1.57079632679, 0, 3.14159265359]  RotationSequenceAnglesUnits=rad  RotationMatrix=[1 0 0; 0 1 0; 0 0 1]
  F : PMIOPort  Side=Left
  F1 : PMIOPort  Port=2  Side=Right
  connections:
  Inertia/RConn1 -- InertiaOriginTransform/RConn1
  InertiaOriginTransform/LConn1 -- ReferenceFrame/RConn1 -- iiwa_joint_2_AxisInvTransform/LConn1 -- iiwa_joint_3_OriginTransform/LConn1 -- VisualOriginTransform/LConn1
  Visual/RConn1 -- VisualOriginTransform/RConn1
  iiwa_joint_2_AxisInvTransform/RConn1 -- F/RConn1
  iiwa_joint_3_AxisTransform/RConn1 -- F1/RConn1
  iiwa_joint_3_AxisTransform/LConn1 -- iiwa_joint_3_OriginTransform/RConn1

== system KUKA_coupled/Space Manipulator1/joint//link3/iiwa_link_3 ==
  Inertia : sm_lib/Body Elements/Inertia  InertiaType=Custom  Mass=4.05623  MassUnits=kg  CenterOfMass=[0, 0, 0]  CenterOfMassUnits=m  MomentsOfInertia=[0.03204, 0.009719999999999999, 0.03042]  MomentsOfInertiaUnits=kg*m^2  ProductsOfInertia=[0.006227, 0, 0]  ProductsOfInertiaUnits=kg*m^2  GraphicType=None  MarkerShape=Inertia  MarkerSize=20  GraphicVisPropType=SimpleVisualProperties  GraphicDiffuseColor=[0.5 0.5 0.5]  GraphicSpecularColor=[0.5 0.5 0.5 1.0]  GraphicAmbientColor=[0.15 0.15 0.15 1.0]  GraphicEmissiveColor=[0.0 0.0 0.0 1.0]  GraphicShininess=75  GraphicOpacity=1.0
  InertiaOriginTransform : sm_lib/Frames and Transforms/Rigid Transform  TranslationMethod=Cartesian  TranslationStandardOffset=0  TranslationLengthUnit=m  TranslationStandardAxis=+Z  TranslationCartesianOffset=[0, 0.03, 0.13]  TranslationROffset=0  TranslationROffsetUnits=m  TranslationZOffset=0  TranslationZOffsetUnits=m  TranslationThetaOffset=0  TranslationThetaOffsetUnits=deg  RotationMethod=RotationSequence  RotationAngleUnits=deg  RotationStandardAxis=+Z  RotationAngle=0.0  RotationArbitraryAxis=[0 0 1]  FollAlignAxisA=+X  BaseAlignAxisA=+Y  FollAlignAxisB=+Y  BaseAlignAxisB=+Z  RotationSequenceAxes=BaseAxes  RotationSequence=XYZ  RotationSequenceAngles=[0, 0, 0]  RotationSequenceAnglesUnits=rad  RotationMatrix=[1 0 0; 0 1 0; 0 0 1]
  ReferenceFrame : sm_lib/Frames and Transforms/Reference Frame
  Visual : sm_lib/Body Elements/File Solid  ExtGeomFileName=iiwa_description/meshes/iiwa7/visual/link_3.stl  UnitType=Custom  ExtGeomFileUnits=m  StepReaderType=HEX  ExportConvexHullGeometry=off  InertiaType=Custom  Mass=0  MassUnits=kg  CenterOfMass=[0, 0, 0]  CenterOfMassUnits=m  MomentsOfInertia=[0, 0, 0]  MomentsOfInertiaUnits=kg*m^2  ProductsOfInertia=[0, 0, 0]  ProductsOfInertiaUnits=kg*m^2  BasedOnType=DensityFromFile  Density=1000  DensityUnits=kg/m^3  DoExposeReferenceFrame=on  SerializedFrames=<Frames/>  GraphicType=FromGeometry  MarkerShape=Sphere  MarkerSize=10  GraphicVisPropType=SimpleVisualProperties  GraphicDiffuseColor=[1, 0.423529411765, 0.0392156862745]  GraphicSpecularColor=[0.5 0.5 0.5 1.0]  GraphicAmbientColor=[0.15 0.15 0.15 1.0]  GraphicEmissiveColor=[0.0 0.0 0.0 1.0]  GraphicShininess=75  GraphicOpacity=1
  VisualOriginTransform : sm_lib/Frames and Transforms/Rigid Transform  TranslationMethod=Cartesian  TranslationStandardOffset=0  TranslationLengthUnit=m  TranslationStandardAxis=+Z  TranslationCartesianOffset=[0, 0, -0.026]  TranslationROffset=0  TranslationROffsetUnits=m  TranslationZOffset=0  TranslationZOffsetUnits=m  TranslationThetaOffset=0  TranslationThetaOffsetUnits=deg  RotationMethod=RotationSequence  RotationAngleUnits=deg  RotationStandardAxis=+Z  RotationAngle=0.0  RotationArbitraryAxis=[0 0 1]  FollAlignAxisA=+X  BaseAlignAxisA=+Y  FollAlignAxisB=+Y  BaseAlignAxisB=+Z  RotationSequenceAxes=BaseAxes  RotationSequence=XYZ  RotationSequenceAngles=[0, 0, 0]  RotationSequenceAnglesUnits=rad  RotationMatrix=[1 0 0; 0 1 0; 0 0 1]
  iiwa_joint_3_AxisInvTransform : sm_lib/Frames and Transforms/Rigid Transform  TranslationMethod=Cartesian  TranslationStandardOffset=0  TranslationLengthUnit=m  TranslationStandardAxis=+Z  TranslationCartesianOffset=[0, 0, 0]  TranslationROffset=0  TranslationROffsetUnits=m  TranslationZOffset=0  TranslationZOffsetUnits=m  TranslationThetaOffset=0  TranslationThetaOffsetUnits=deg  RotationMethod=ArbitraryAxis  RotationAngleUnits=rad  RotationStandardAxis=+Z  RotationAngle=0  RotationArbitraryAxis=[1, 0, 0]  FollAlignAxisA=+X  BaseAlignAxisA=+Y  FollAlignAxisB=+Y  BaseAlignAxisB=+Z  RotationSequenceAxes=FollowerAxes  RotationSequence=XYX  RotationSequenceAngles=[0 0 0]  RotationSequenceAnglesUnits=deg  RotationMatrix=[1 0 0; 0 1 0; 0 0 1]
  iiwa_joint_4_AxisTransform : sm_lib/Frames and Transforms/Rigid Transform  TranslationMethod=Cartesian  TranslationStandardOffset=0  TranslationLengthUnit=m  TranslationStandardAxis=+Z  TranslationCartesianOffset=[0, 0, 0]  TranslationROffset=0  TranslationROffsetUnits=m  TranslationZOffset=0  TranslationZOffsetUnits=m  TranslationThetaOffset=0  TranslationThetaOffsetUnits=deg  RotationMethod=ArbitraryAxis  RotationAngleUnits=rad  RotationStandardAxis=+Z  RotationAngle=0  RotationArbitraryAxis=[1, 0, 0]  FollAlignAxisA=+X  BaseAlignAxisA=+Y  FollAlignAxisB=+Y  BaseAlignAxisB=+Z  RotationSequenceAxes=FollowerAxes  RotationSequence=XYX  RotationSequenceAngles=[0 0 0]  RotationSequenceAnglesUnits=deg  RotationMatrix=[1 0 0; 0 1 0; 0 0 1]
  iiwa_joint_4_OriginTransform : sm_lib/Frames and Transforms/Rigid Transform  TranslationMethod=Cartesian  TranslationStandardOffset=0  TranslationLengthUnit=m  TranslationStandardAxis=+Z  TranslationCartesianOffset=[0, 0, 0.19]  TranslationROffset=0  TranslationROffsetUnits=m  TranslationZOffset=0  TranslationZOffsetUnits=m  TranslationThetaOffset=0  TranslationThetaOffsetUnits=deg  RotationMethod=RotationSequence  RotationAngleUnits=deg  RotationStandardAxis=+Z  RotationAngle=0.0  RotationArbitraryAxis=[0 0 1]  FollAlignAxisA=+X  BaseAlignAxisA=+Y  FollAlignAxisB=+Y  BaseAlignAxisB=+Z  RotationSequenceAxes=BaseAxes  RotationSequence=XYZ  RotationSequenceAngles=[1.57079632679, 0, 0]  RotationSequenceAnglesUnits=rad  RotationMatrix=[1 0 0; 0 1 0; 0 0 1]
  F : PMIOPort  Side=Left
  F1 : PMIOPort  Port=2  Side=Right
  connections:
  Inertia/RConn1 -- InertiaOriginTransform/RConn1
  InertiaOriginTransform/LConn1 -- iiwa_joint_3_AxisInvTransform/LConn1 -- iiwa_joint_4_OriginTransform/LConn1 -- VisualOriginTransform/LConn1 -- ReferenceFrame/RConn1
  Visual/RConn1 -- VisualOriginTransform/RConn1
  iiwa_joint_3_AxisInvTransform/RConn1 -- F/RConn1
  iiwa_joint_4_AxisTransform/RConn1 -- F1/RConn1
  iiwa_joint_4_AxisTransform/LConn1 -- iiwa_joint_4_OriginTransform/RConn1
